simulink model "rfsoc4x2_ospfb_128"  (R2021a)
settings: Solver=VariableStepAuto  StartTime=0.0  StopTime=2048  RelTol=1e-3
undefined symbols (not defined in the file): pfb_coeff_gen_calc
libraries: xbsIndex_r4 x37092, casper_library_delays x737, casper_library_misc x68, xps_library x1
(part 274 of 339)

== system rfsoc4x2_ospfb_128/fft_wideband_real1/fft_biplex_real_4x/biplex_core/fft_stage_3/butterfly_direct/bus_convert ==
  din : Inport
  bussify : Subsystem  AncestorBlock=casper_library_flow_control/bus_create  mask(bus_create){inputNum=16}
      mask prompts: inputNum "Number of inputs:"
      mask init:
      | bus_create_init(gcb,...
      |     'inputNum', inputNum);
  conv1 : Subsystem  AncestorBlock=casper_library_misc/convert_of  mask(convert_of){bit_width_i=21, binary_point_i=18, bit_width_o=18, binary_point_o=17, csp_latency=3, overflow=Wrap, quantization=Round  (unbiased: +/- Inf)}
      mask prompts: bit_width_i "Bit Width In"; binary_point_i "Binary Point In"; bit_width_o "Bit Width Out"; binary_point_o "Binary Point Out"; csp_latency "Latency"; overflow "Overflow Behaviour"; quantization "Quantization Behaviour"
      mask help:
      | Converts from one 2's complement bit-width
      | and/or binary point position to another.
      | Includes underflow/overflow indicator.
      mask init: same as rfsoc4x2_ospfb_128/fft2/fft_direct/butterfly0_0/bus_convert/conv1
      settings: AttributesFormatString=[21,18]->[18,17]
      mask TypeOptions overflow: Wrap | Saturate | Error
      mask TypeOptions quantization: Truncate | Round  (unbiased: +/- Inf) | Round  (unbiased: even values)
  conv10 : Subsystem  AncestorBlock=casper_library_misc/convert_of  mask(convert_of){bit_width_i=21, binary_point_i=18, bit_width_o=18, binary_point_o=17, csp_latency=3, overflow=Wrap, quantization=Round  (unbiased: +/- Inf)}
      mask prompts: bit_width_i "Bit Width In"; binary_point_i "Binary Point In"; bit_width_o "Bit Width Out"; binary_point_o "Binary Point Out"; csp_latency "Latency"; overflow "Overflow Behaviour"; quantization "Quantization Behaviour"
      mask help:
      | Converts from one 2's complement bit-width
      | and/or binary point position to another.
      | Includes underflow/overflow indicator.
      mask init: same as rfsoc4x2_ospfb_128/fft2/fft_direct/butterfly0_0/bus_convert/conv1
      settings: AttributesFormatString=[21,18]->[18,17]
      mask TypeOptions overflow: Wrap | Saturate | Error
      mask TypeOptions quantization: Truncate | Round  (unbiased: +/- Inf) | Round  (unbiased: even values)
  conv11 : Subsystem  AncestorBlock=casper_library_misc/convert_of  mask(convert_of){bit_width_i=21, binary_point_i=18, bit_width_o=18, binary_point_o=17, csp_latency=3, overflow=Wrap, quantization=Round  (unbiased: +/- Inf)}
      mask prompts: bit_width_i "Bit Width In"; binary_point_i "Binary Point In"; bit_width_o "Bit Width Out"; binary_point_o "Binary Point Out"; csp_latency "Latency"; overflow "Overflow Behaviour"; quantization "Quantization Behaviour"
      mask help:
      | Converts from one 2's complement bit-width
      | and/or binary point position to another.
      | Includes underflow/overflow indicator.
      mask init: same as rfsoc4x2_ospfb_128/fft2/fft_direct/butterfly0_0/bus_convert/conv1
      settings: AttributesFormatString=[21,18]->[18,17]
      mask TypeOptions overflow: Wrap | Saturate | Error
      mask TypeOptions quantization: Truncate | Round  (unbiased: +/- Inf) | Round  (unbiased: even values)
  conv12 : Subsystem  AncestorBlock=casper_library_misc/convert_of  mask(convert_of){bit_width_i=21, binary_point_i=18, bit_width_o=18, binary_point_o=17, csp_latency=3, overflow=Wrap, quantization=Round  (unbiased: +/- Inf)}
      mask prompts: bit_width_i "Bit Width In"; binary_point_i "Binary Point In"; bit_width_o "Bit Width Out"; binary_point_o "Binary Point Out"; csp_latency "Latency"; overflow "Overflow Behaviour"; quantization "Quantization Behaviour"
      mask help:
      | Converts from one 2's complement bit-width
      | and/or binary point position to another.
      | Includes underflow/overflow indicator.
      mask init: same as rfsoc4x2_ospfb_128/fft2/fft_direct/butterfly0_0/bus_convert/conv1
      settings: AttributesFormatString=[21,18]->[18,17]
      mask TypeOptions overflow: Wrap | Saturate | Error
      mask TypeOptions quantization: Truncate | Round  (unbiased: +/- Inf) | Round  (unbiased: even values)
  conv13 : Subsystem  AncestorBlock=casper_library_misc/convert_of  mask(convert_of){bit_width_i=21, binary_point_i=18, bit_width_o=18, binary_point_o=17, csp_latency=3, overflow=Wrap, quantization=Round  (unbiased: +/- Inf)}
      mask prompts: bit_width_i "Bit Width In"; binary_point_i "Binary Point In"; bit_width_o "Bit Width Out"; binary_point_o "Binary Point Out"; csp_latency "Latency"; overflow "Overflow Behaviour"; quantization "Quantization Behaviour"
      mask help:
      | Converts from one 2's complement bit-width
      | and/or binary point position to another.
      | Includes underflow/overflow indicator.
      mask init: same as rfsoc4x2_ospfb_128/fft2/fft_direct/butterfly0_0/bus_convert/conv1
      settings: AttributesFormatString=[21,18]->[18,17]
      mask TypeOptions overflow: Wrap | Saturate | Error
      mask TypeOptions quantization: Truncate | Round  (unbiased: +/- Inf) | Round  (unbiased: even values)
  conv14 : Subsystem  AncestorBlock=casper_library_misc/convert_of  mask(convert_of){bit_width_i=21, binary_point_i=18, bit_width_o=18, binary_point_o=17, csp_latency=3, overflow=Wrap, quantization=Round  (unbiased: +/- Inf)}
      mask prompts: bit_width_i "Bit Width In"; binary_point_i "Binary Point In"; bit_width_o "Bit Width Out"; binary_point_o "Binary Point Out"; csp_latency "Latency"; overflow "Overflow Behaviour"; quantization "Quantization Behaviour"
      mask help:
      | Converts from one 2's complement bit-width
      | and/or binary point position to another.
      | Includes underflow/overflow indicator.
      mask init: same as rfsoc4x2_ospfb_128/fft2/fft_direct/butterfly0_0/bus_convert/conv1
      settings: AttributesFormatString=[21,18]->[18,17]
      mask TypeOptions overflow: Wrap | Saturate | Error
      mask TypeOptions quantization: Truncate | Round  (unbiased: +/- Inf) | Round  (unbiased: even values)
  conv15 : Subsystem  AncestorBlock=casper_library_misc/convert_of  mask(convert_of){bit_width_i=21, binary_point_i=18, bit_width_o=18, binary_point_o=17, csp_latency=3, overflow=Wrap, quantization=Round  (unbiased: +/- Inf)}
      mask prompts: bit_width_i "Bit Width In"; binary_point_i "Binary Point In"; bit_width_o "Bit Width Out"; binary_point_o "Binary Point Out"; csp_latency "Latency"; overflow "Overflow Behaviour"; quantization "Quantization Behaviour"
      mask help:
      | Converts from one 2's complement bit-width
      | and/or binary point position to another.
      | Includes underflow/overflow indicator.
      mask init: same as rfsoc4x2_ospfb_128/fft2/fft_direct/butterfly0_0/bus_convert/conv1
      settings: AttributesFormatString=[21,18]->[18,17]
      mask TypeOptions overflow: Wrap | Saturate | Error
      mask TypeOptions quantization: Truncate | Round  (unbiased: +/- Inf) | Round  (unbiased: even values)
  conv16 : Subsystem  AncestorBlock=casper_library_misc/convert_of  mask(convert_of){bit_width_i=21, binary_point_i=18, bit_width_o=18, binary_point_o=17, csp_latency=3, overflow=Wrap, quantization=Round  (unbiased: +/- Inf)}
      mask prompts: bit_width_i "Bit Width In"; binary_point_i "Binary Point In"; bit_width_o "Bit Width Out"; binary_point_o "Binary Point Out"; csp_latency "Latency"; overflow "Overflow Behaviour"; quantization "Quantization Behaviour"
      mask help:
      | Converts from one 2's complement bit-width
      | and/or binary point position to another.
      | Includes underflow/overflow indicator.
      mask init: same as rfsoc4x2_ospfb_128/fft2/fft_direct/butterfly0_0/bus_convert/conv1
      settings: AttributesFormatString=[21,18]->[18,17]
      mask TypeOptions overflow: Wrap | Saturate | Error
      mask TypeOptions quantization: Truncate | Round  (unbiased: +/- Inf) | Round  (unbiased: even values)
  conv2 : Subsystem  AncestorBlock=casper_library_misc/convert_of  mask(convert_of){bit_width_i=21, binary_point_i=18, bit_width_o=18, binary_point_o=17, csp_latency=3, overflow=Wrap, quantization=Round  (unbiased: +/- Inf)}
      mask prompts: bit_width_i "Bit Width In"; binary_point_i "Binary Point In"; bit_width_o "Bit Width Out"; binary_point_o "Binary Point Out"; csp_latency "Latency"; overflow "Overflow Behaviour"; quantization "Quantization Behaviour"
      mask help:
      | Converts from one 2's complement bit-width
      | and/or binary point position to another.
      | Includes underflow/overflow indicator.
      mask init: same as rfsoc4x2_ospfb_128/fft2/fft_direct/butterfly0_0/bus_convert/conv1
      settings: AttributesFormatString=[21,18]->[18,17]
      mask TypeOptions overflow: Wrap | Saturate | Error
      mask TypeOptions quantization: Truncate | Round  (unbiased: +/- Inf) | Round  (unbiased: even values)
  conv3 : Subsystem  AncestorBlock=casper_library_misc/convert_of  mask(convert_of){bit_width_i=21, binary_point_i=18, bit_width_o=18, binary_point_o=17, csp_latency=3, overflow=Wrap, quantization=Round  (unbiased: +/- Inf)}
      mask prompts: bit_width_i "Bit Width In"; binary_point_i "Binary Point In"; bit_width_o "Bit Width Out"; binary_point_o "Binary Point Out"; csp_latency "Latency"; overflow "Overflow Behaviour"; quantization "Quantization Behaviour"
      mask help:
      | Converts from one 2's complement bit-width
      | and/or binary point position to another.
      | Includes underflow/overflow indicator.
      mask init: same as rfsoc4x2_ospfb_128/fft2/fft_direct/butterfly0_0/bus_convert/conv1
      settings: AttributesFormatString=[21,18]->[18,17]
      mask TypeOptions overflow: Wrap | Saturate | Error
      mask TypeOptions quantization: Truncate | Round  (unbiased: +/- Inf) | Round  (unbiased: even values)
  conv4 : Subsystem  AncestorBlock=casper_library_misc/convert_of  mask(convert_of){bit_width_i=21, binary_point_i=18, bit_width_o=18, binary_point_o=17, csp_latency=3, overflow=Wrap, quantization=Round  (unbiased: +/- Inf)}
      mask prompts: bit_width_i "Bit Width In"; binary_point_i "Binary Point In"; bit_width_o "Bit Width Out"; binary_point_o "Binary Point Out"; csp_latency "Latency"; overflow "Overflow Behaviour"; quantization "Quantization Behaviour"
      mask help:
      | Converts from one 2's complement bit-width
      | and/or binary point position to another.
      | Includes underflow/overflow indicator.
      mask init: same as rfsoc4x2_ospfb_128/fft2/fft_direct/butterfly0_0/bus_convert/conv1
      settings: AttributesFormatString=[21,18]->[18,17]
      mask TypeOptions overflow: Wrap | Saturate | Error
      mask TypeOptions quantization: Truncate | Round  (unbiased: +/- Inf) | Round  (unbiased: even values)
  conv5 : Subsystem  AncestorBlock=casper_library_misc/convert_of  mask(convert_of){bit_width_i=21, binary_point_i=18, bit_width_o=18, binary_point_o=17, csp_latency=3, overflow=Wrap, quantization=Round  (unbiased: +/- Inf)}
      mask prompts: bit_width_i "Bit Width In"; binary_point_i "Binary Point In"; bit_width_o "Bit Width Out"; binary_point_o "Binary Point Out"; csp_latency "Latency"; overflow "Overflow Behaviour"; quantization "Quantization Behaviour"
      mask help:
      | Converts from one 2's complement bit-width
      | and/or binary point position to another.
      | Includes underflow/overflow indicator.
      mask init: same as rfsoc4x2_ospfb_128/fft2/fft_direct/butterfly0_0/bus_convert/conv1
      settings: AttributesFormatString=[21,18]->[18,17]
      mask TypeOptions overflow: Wrap | Saturate | Error
      mask TypeOptions quantization: Truncate | Round  (unbiased: +/- Inf) | Round  (unbiased: even values)
  conv6 : Subsystem  AncestorBlock=casper_library_misc/convert_of  mask(convert_of){bit_width_i=21, binary_point_i=18, bit_width_o=18, binary_point_o=17, csp_latency=3, overflow=Wrap, quantization=Round  (unbiased: +/- Inf)}
      mask prompts: bit_width_i "Bit Width In"; binary_point_i "Binary Point In"; bit_width_o "Bit Width Out"; binary_point_o "Binary Point Out"; csp_latency "Latency"; overflow "Overflow Behaviour"; quantization "Quantization Behaviour"
      mask help:
      | Converts from one 2's complement bit-width
      | and/or binary point position to another.
      | Includes underflow/overflow indicator.
      mask init: same as rfsoc4x2_ospfb_128/fft2/fft_direct/butterfly0_0/bus_convert/conv1
      settings: AttributesFormatString=[21,18]->[18,17]
      mask TypeOptions overflow: Wrap | Saturate | Error
      mask TypeOptions quantization: Truncate | Round  (unbiased: +/- Inf) | Round  (unbiased: even values)
  conv7 : Subsystem  AncestorBlock=casper_library_misc/convert_of  mask(convert_of){bit_width_i=21, binary_point_i=18, bit_width_o=18, binary_point_o=17, csp_latency=3, overflow=Wrap, quantization=Round  (unbiased: +/- Inf)}
      mask prompts: bit_width_i "Bit Width In"; binary_point_i "Binary Point In"; bit_width_o "Bit Width Out"; binary_point_o "Binary Point Out"; csp_latency "Latency"; overflow "Overflow Behaviour"; quantization "Quantization Behaviour"
      mask help:
      | Converts from one 2's complement bit-width
      | and/or binary point position to another.
      | Includes underflow/overflow indicator.
      mask init: same as rfsoc4x2_ospfb_128/fft2/fft_direct/butterfly0_0/bus_convert/conv1
      settings: AttributesFormatString=[21,18]->[18,17]
      mask TypeOptions overflow: Wrap | Saturate | Error
      mask TypeOptions quantization: Truncate | Round  (unbiased: +/- Inf) | Round  (unbiased: even values)
  conv8 : Subsystem  AncestorBlock=casper_library_misc/convert_of  mask(convert_of){bit_width_i=21, binary_point_i=18, bit_width_o=18, binary_point_o=17, csp_latency=3, overflow=Wrap, quantization=Round  (unbiased: +/- Inf)}
      mask prompts: bit_width_i "Bit Width In"; binary_point_i "Binary Point In"; bit_width_o "Bit Width Out"; binary_point_o "Binary Point Out"; csp_latency "Latency"; overflow "Overflow Behaviour"; quantization "Quantization Behaviour"
      mask help:
      | Converts from one 2's complement bit-width
      | and/or binary point position to another.
      | Includes underflow/overflow indicator.
      mask init: same as rfsoc4x2_ospfb_128/fft2/fft_direct/butterfly0_0/bus_convert/conv1
      settings: AttributesFormatString=[21,18]->[18,17]
      mask TypeOptions overflow: Wrap | Saturate | Error
      mask TypeOptions quantization: Truncate | Round  (unbiased: +/- Inf) | Round  (unbiased: even values)
  conv9 : Subsystem  AncestorBlock=casper_library_misc/convert_of  mask(convert_of){bit_width_i=21, binary_point_i=18, bit_width_o=18, binary_point_o=17, csp_latency=3, overflow=Wrap, quantization=Round  (unbiased: +/- Inf)}
      mask prompts: bit_width_i "Bit Width In"; binary_point_i "Binary Point In"; bit_width_o "Bit Width Out"; binary_point_o "Binary Point Out"; csp_latency "Latency"; overflow "Overflow Behaviour"; quantization "Quantization Behaviour"
      mask help:
      | Converts from one 2's complement bit-width
      | and/or binary point position to another.
      | Includes underflow/overflow indicator.
      mask init: same as rfsoc4x2_ospfb_128/fft2/fft_direct/butterfly0_0/bus_convert/conv1
      settings: AttributesFormatString=[21,18]->[18,17]
      mask TypeOptions overflow: Wrap | Saturate | Error
      mask TypeOptions quantization: Truncate | Round  (unbiased: +/- Inf) | Round  (unbiased: even values)
  debus : Subsystem  AncestorBlock=casper_library_flow_control/bus_expand  mask(bus_expand){mode=divisions of arbitrary size, outputNum=2, outputWidth=[21 21 21 21 21 21 21 21 21 21 21 21 21 21 21 21], outputBinaryPt=[18 18 18 18 18 18 18 18 18 18 18 18 18 18 18 18], outputArithmeticType=[1 1 1 1 1 1 1 1 1 1 1 1 1 1 1 1], show_format=on, outputToWorkspace=off, variablePrefix=, outputToModelAsWell=on}
      mask prompts: outputNum "Number of outputs:"; outputWidth "Output width:"; outputBinaryPt "Output binary point position:"; outputArithmeticType "Output arithmetic type (ufix=0, fix=1, bool=2):"; show_format "Print format string?"; outputToWorkspace "Output to workspace?"; variablePrefix "Variable name prefix:"; outputToModelAsWell "Output to model as well?"
      mask help:
      | Expands a 'bus' made using a bus_create or Xilinx
      | concat block.
      | The input will be divided into the specified number
      | of outputs with the specified arithmetic types.
      | Divisions are made from most significant bit.
      mask init: same as rfsoc4x2_ospfb_128/bus_expand1
      settings: AttributesFormatString=16 outputs: f21.18,f21.18,f21.18,f21.18,f21.18,f21.18,f21.18,f21.18,f21.18,f21.18,f21.18,f21.18,f21.18,f21.18,f21.18,f21.18,
      mask TypeOptions mode: divisions of equal size | divisions of arbitrary size
      mask Callback mode: %bus_expand_callback();
      mask Callback outputWidth: %bus_expand_callback();
      mask Callback outputToWorkspace: %bus_expand_callback();
  of_bussify : Subsystem  AncestorBlock=casper_library_flow_control/bus_create  mask(bus_create){inputNum=16}
      mask prompts: inputNum "Number of inputs:"
      mask init:
      | bus_create_init(gcb,...
      |     'inputNum', inputNum);
  dout : Outport
  overflow : Outport  Port=2
  wires:
  of_bussify/1(bus_out) -> overflow/1
  bussify/1(bus_out) -> dout/1
  conv16/2(of) -> of_bussify/16(in16)
  conv15/2(of) -> of_bussify/15(in15)
  conv14/2(of) -> of_bussify/14(in14)
  conv13/2(of) -> of_bussify/13(in13)
  conv12/2(of) -> of_bussify/12(in12)
  conv11/2(of) -> of_bussify/11(in11)
  conv10/2(of) -> of_bussify/10(in10)
  conv9/2(of) -> of_bussify/9(in9)
  conv8/2(of) -> of_bussify/8(in8)
  conv7/2(of) -> of_bussify/7(in7)
  conv6/2(of) -> of_bussify/6(in6)
  conv5/2(of) -> of_bussify/5(in5)
  conv4/2(of) -> of_bussify/4(in4)
  conv3/2(of) -> of_bussify/3(in3)
  conv2/2(of) -> of_bussify/2(in2)
  conv1/2(of) -> of_bussify/1(in1)
  conv16/1(dout) -> bussify/16(in16)
  conv15/1(dout) -> bussify/15(in15)
  conv14/1(dout) -> bussify/14(in14)
  conv13/1(dout) -> bussify/13(in13)
  conv12/1(dout) -> bussify/12(in12)
  conv11/1(dout) -> bussify/11(in11)
  conv10/1(dout) -> bussify/10(in10)
  conv9/1(dout) -> bussify/9(in9)
  conv8/1(dout) -> bussify/8(in8)
  conv7/1(dout) -> bussify/7(in7)
  conv6/1(dout) -> bussify/6(in6)
  conv5/1(dout) -> bussify/5(in5)
  conv4/1(dout) -> bussify/4(in4)
  conv3/1(dout) -> bussify/3(in3)
  conv2/1(dout) -> bussify/2(in2)
  conv1/1(dout) -> bussify/1(in1)
  debus/16(lsb_out1) -> conv16/1(din)
  debus/15(out2) -> conv15/1(din)
  debus/14(out3) -> conv14/1(din)
  debus/13(out4) -> conv13/1(din)
  debus/12(out5) -> conv12/1(din)
  debus/11(out6) -> conv11/1(din)
  debus/10(out7) -> conv10/1(din)
  debus/9(out8) -> conv9/1(din)
  debus/8(out9) -> conv8/1(din)
  debus/7(out10) -> conv7/1(din)
  debus/6(out11) -> conv6/1(din)
  debus/5(out12) -> conv5/1(din)
  debus/4(out13) -> conv4/1(din)
  debus/3(out14) -> conv3/1(din)
  debus/2(out15) -> conv2/1(din)
  debus/1(msb_out16) -> conv1/1(din)
  din/1 -> debus/1(bus_in)

== system rfsoc4x2_ospfb_128/fft_wideband_real1/fft_biplex_real_4x/biplex_core/fft_stage_3/butterfly_direct/bus_expand ==
  bus_in : Inport
  reinterpret1 : xbsIndex_r4/Reinterpret  force_arith_type=on  arith_type=Unsigned  force_bin_pt=on  bin_pt=0  block_type=reinterpret
  reinterpret2 : xbsIndex_r4/Reinterpret  force_arith_type=on  arith_type=Unsigned  force_bin_pt=on  bin_pt=0  block_type=reinterpret
  slice1 : xbsIndex_r4/Slice  nbits=144  boolean_output=off  mode=Upper Bit Location + Width  bit1=-144  base1=MSB of Input  bit0=0  base0=LSB of Input  dbl_ovrd=off  block_type=slice
  slice2 : xbsIndex_r4/Slice  nbits=144  boolean_output=off  mode=Upper Bit Location + Width  bit1=0  base1=MSB of Input  bit0=0  base0=LSB of Input  dbl_ovrd=off  block_type=slice
  msb_out2 : Outport  VectorParamsAs1DForOutWhenUnconnected=off
  lsb_out1 : Outport  Port=2  VectorParamsAs1DForOutWhenUnconnected=off
  wires:
  reinterpret1/1 -> lsb_out1/1
  slice1/1 -> reinterpret1/1
  reinterpret2/1 -> msb_out2/1
  slice2/1 -> reinterpret2/1
  bus_in/1 -> slice1/1, slice2/1

== system rfsoc4x2_ospfb_128/fft_wideband_real1/fft_biplex_real_4x/biplex_core/fft_stage_3/butterfly_direct/bus_norm0 ==
  din : Inport
  bussify : Subsystem  AncestorBlock=casper_library_flow_control/bus_create  mask(bus_create){inputNum=16}
      mask prompts: inputNum "Number of inputs:"
      mask init:
      | bus_create_init(gcb,...
      |     'inputNum', inputNum);
  conv{1..16} (16 alike) : xbsIndex_r4/Convert  gui_display_data_type=Fixed-point  arith_type="Signed  (2's comp)"  n_bits=21  bin_pt=18  float_type=Single  exp_bits=8  fraction_bits=24  quantization=Truncate  overflow=Wrap  en=off  latency=0  pipeline=on  dbl_ovrd=off  block_type=convert
  debus : Subsystem  AncestorBlock=casper_library_flow_control/bus_expand  mask(bus_expand){mode=divisions of arbitrary size, outputNum=2, outputWidth=[20 20 20 20 20 20 20 20 20 20 20 20 20 20 20 20], outputBinaryPt=[17 17 17 17 17 17 17 17 17 17 17 17 17 17 17 17], outputArithmeticType=[1 1 1 1 1 1 1 1 1 1 1 1 1 1 1 1], show_format=on, outputToWorkspace=off, variablePrefix=, outputToModelAsWell=on}
      mask prompts: outputNum "Number of outputs:"; outputWidth "Output width:"; outputBinaryPt "Output binary point position:"; outputArithmeticType "Output arithmetic type (ufix=0, fix=1, bool=2):"; show_format "Print format string?"; outputToWorkspace "Output to workspace?"; variablePrefix "Variable name prefix:"; outputToModelAsWell "Output to model as well?"
      mask help:
      | Expands a 'bus' made using a bus_create or Xilinx
      | concat block.
      | The input will be divided into the specified number
      | of outputs with the specified arithmetic types.
      | Divisions are made from most significant bit.
      mask init: same as rfsoc4x2_ospfb_128/bus_expand1
      settings: AttributesFormatString=16 outputs: f20.17,f20.17,f20.17,f20.17,f20.17,f20.17,f20.17,f20.17,f20.17,f20.17,f20.17,f20.17,f20.17,f20.17,f20.17,f20.17,
      mask TypeOptions mode: divisions of equal size | divisions of arbitrary size
      mask Callback mode: %bus_expand_callback();
      mask Callback outputWidth: %bus_expand_callback();
      mask Callback outputToWorkspace: %bus_expand_callback();
  dout : Outport
  wires:
  bussify/1(bus_out) -> dout/1
  conv16/1 -> bussify/16(in16)
  conv15/1 -> bussify/15(in15)
  conv14/1 -> bussify/14(in14)
  conv13/1 -> bussify/13(in13)
  conv12/1 -> bussify/12(in12)
  conv11/1 -> bussify/11(in11)
  conv10/1 -> bussify/10(in10)
  conv9/1 -> bussify/9(in9)
  conv8/1 -> bussify/8(in8)
  conv7/1 -> bussify/7(in7)
  conv6/1 -> bussify/6(in6)
  conv5/1 -> bussify/5(in5)
  conv4/1 -> bussify/4(in4)
  conv3/1 -> bussify/3(in3)
  conv2/1 -> bussify/2(in2)
  conv1/1 -> bussify/1(in1)
  debus/16(lsb_out1) -> conv16/1
  debus/15(out2) -> conv15/1
  debus/14(out3) -> conv14/1
  debus/13(out4) -> conv13/1
  debus/12(out5) -> conv12/1
  debus/11(out6) -> conv11/1
  debus/10(out7) -> conv10/1
  debus/9(out8) -> conv9/1
  debus/8(out9) -> conv8/1
  debus/7(out10) -> conv7/1
  debus/6(out11) -> conv6/1
  debus/5(out12) -> conv5/1
  debus/4(out13) -> conv4/1
  debus/3(out14) -> conv3/1
  debus/2(out15) -> conv2/1
  debus/1(msb_out16) -> conv1/1
  din/1 -> debus/1(bus_in)

== system rfsoc4x2_ospfb_128/fft_wideband_real1/fft_biplex_real_4x/biplex_core/fft_stage_3/butterfly_direct/bus_norm1 ==
  din : Inport
  bussify : Subsystem  AncestorBlock=casper_library_flow_control/bus_create  mask(bus_create){inputNum=16}
      mask prompts: inputNum "Number of inputs:"
      mask init:
      | bus_create_init(gcb,...
      |     'inputNum', inputNum);
  conv{1..16} (16 alike) : xbsIndex_r4/Convert  gui_display_data_type=Fixed-point  arith_type="Signed  (2's comp)"  n_bits=21  bin_pt=18  float_type=Single  exp_bits=8  fraction_bits=24  quantization=Truncate  overflow=Wrap  en=off  latency=0  pipeline=on  dbl_ovrd=off  block_type=convert
  debus : Subsystem  AncestorBlock=casper_library_flow_control/bus_expand  mask(bus_expand){mode=divisions of arbitrary size, outputNum=2, outputWidth=[20 20 20 20 20 20 20 20 20 20 20 20 20 20 20 20], outputBinaryPt=[18 18 18 18 18 18 18 18 18 18 18 18 18 18 18 18], outputArithmeticType=[1 1 1 1 1 1 1 1 1 1 1 1 1 1 1 1], show_format=on, outputToWorkspace=off, variablePrefix=, outputToModelAsWell=on}
      mask prompts: outputNum "Number of outputs:"; outputWidth "Output width:"; outputBinaryPt "Output binary point position:"; outputArithmeticType "Output arithmetic type (ufix=0, fix=1, bool=2):"; show_format "Print format string?"; outputToWorkspace "Output to workspace?"; variablePrefix "Variable name prefix:"; outputToModelAsWell "Output to model as well?"
      mask help:
      | Expands a 'bus' made using a bus_create or Xilinx
      | concat block.
      | The input will be divided into the specified number
      | of outputs with the specified arithmetic types.
      | Divisions are made from most significant bit.
      mask init: same as rfsoc4x2_ospfb_128/bus_expand1
      settings: AttributesFormatString=16 outputs: f20.18,f20.18,f20.18,f20.18,f20.18,f20.18,f20.18,f20.18,f20.18,f20.18,f20.18,f20.18,f20.18,f20.18,f20.18,f20.18,
      mask TypeOptions mode: divisions of equal size | divisions of arbitrary size
      mask Callback mode: %bus_expand_callback();
      mask Callback outputWidth: %bus_expand_callback();
      mask Callback outputToWorkspace: %bus_expand_callback();
  dout : Outport
  wires:
  bussify/1(bus_out) -> dout/1
  conv16/1 -> bussify/16(in16)
  conv15/1 -> bussify/15(in15)
  conv14/1 -> bussify/14(in14)
  conv13/1 -> bussify/13(in13)
  conv12/1 -> bussify/12(in12)
  conv11/1 -> bussify/11(in11)
  conv10/1 -> bussify/10(in10)
  conv9/1 -> bussify/9(in9)
  conv8/1 -> bussify/8(in8)
  conv7/1 -> bussify/7(in7)
  conv6/1 -> bussify/6(in6)
  conv5/1 -> bussify/5(in5)
  conv4/1 -> bussify/4(in4)
  conv3/1 -> bussify/3(in3)
  conv2/1 -> bussify/2(in2)
  conv1/1 -> bussify/1(in1)
  debus/16(lsb_out1) -> conv16/1
  debus/15(out2) -> conv15/1
  debus/14(out3) -> conv14/1
  debus/13(out4) -> conv13/1
  debus/12(out5) -> conv12/1
  debus/11(out6) -> conv11/1
  debus/10(out7) -> conv10/1
  debus/9(out8) -> conv9/1
  debus/8(out9) -> conv8/1
  debus/7(out10) -> conv7/1
  debus/6(out11) -> conv6/1
  debus/5(out12) -> conv5/1
  debus/4(out13) -> conv4/1
  debus/3(out14) -> conv3/1
  debus/2(out15) -> conv2/1
  debus/1(msb_out16) -> conv1/1
  din/1 -> debus/1(bus_in)

== system rfsoc4x2_ospfb_128/fft_wideband_real1/fft_biplex_real_4x/biplex_core/fft_stage_3/butterfly_direct/bus_relational ==
  a : Inport
  b : Inport  Port=2
  a_debus : Subsystem  AncestorBlock=casper_library_flow_control/bus_expand  mask(bus_expand){mode=divisions of arbitrary size, outputNum=2, outputWidth=[4], outputBinaryPt=[0], outputArithmeticType=[0], show_format=on, outputToWorkspace=off, variablePrefix=, outputToModelAsWell=on}
      mask prompts: outputNum "Number of outputs:"; outputWidth "Output width:"; outputBinaryPt "Output binary point position:"; outputArithmeticType "Output arithmetic type (ufix=0, fix=1, bool=2):"; show_format "Print format string?"; outputToWorkspace "Output to workspace?"; variablePrefix "Variable name prefix:"; outputToModelAsWell "Output to model as well?"
      mask help:
      | Expands a 'bus' made using a bus_create or Xilinx
      | concat block.
      | The input will be divided into the specified number
      | of outputs with the specified arithmetic types.
      | Divisions are made from most significant bit.
      mask init: same as rfsoc4x2_ospfb_128/bus_expand1
      settings: AttributesFormatString=1 outputs: uf4.0,
      mask TypeOptions mode: divisions of equal size | divisions of arbitrary size
      mask Callback mode: %bus_expand_callback();
      mask Callback outputWidth: %bus_expand_callback();
      mask Callback outputToWorkspace: %bus_expand_callback();
  b_debus : Subsystem  AncestorBlock=casper_library_flow_control/bus_expand  mask(bus_expand){mode=divisions of arbitrary size, outputNum=2, outputWidth=[4  4  4  4], outputBinaryPt=[0  0  0  0], outputArithmeticType=[0  0  0  0], show_format=on, outputToWorkspace=off, variablePrefix=, outputToModelAsWell=on}
      mask prompts: outputNum "Number of outputs:"; outputWidth "Output width:"; outputBinaryPt "Output binary point position:"; outputArithmeticType "Output arithmetic type (ufix=0, fix=1, bool=2):"; show_format "Print format string?"; outputToWorkspace "Output to workspace?"; variablePrefix "Variable name prefix:"; outputToModelAsWell "Output to model as well?"
      mask help:
      | Expands a 'bus' made using a bus_create or Xilinx
      | concat block.
      | The input will be divided into the specified number
      | of outputs with the specified arithmetic types.
      | Divisions are made from most significant bit.
      mask init: same as rfsoc4x2_ospfb_128/bus_expand1
      settings: AttributesFormatString=4 outputs: uf4.0,uf4.0,uf4.0,uf4.0,
      mask TypeOptions mode: divisions of equal size | divisions of arbitrary size
      mask Callback mode: %bus_expand_callback();
      mask Callback outputWidth: %bus_expand_callback();
      mask Callback outputToWorkspace: %bus_expand_callback();
  bussify : Subsystem  AncestorBlock=casper_library_flow_control/bus_create  mask(bus_create){inputNum=4}
      mask prompts: inputNum "Number of inputs:"
      mask init:
      | bus_create_init(gcb,...
      |     'inputNum', inputNum);
  relational{1..4} (4 alike) : xbsIndex_r4/Relational  mode=a!=b  op_type=Bool  en=off  latency=1  dbl_ovrd=off  block_type=relational
  a!=b : Outport
  wires:
  bussify/1(bus_out) -> a!=b/1
  relational4/1 -> bussify/4(in4)
  relational3/1 -> bussify/3(in3)
  relational2/1 -> bussify/2(in2)
  relational1/1 -> bussify/1(in1)
  b_debus/4(lsb_out1) -> relational4/2
  b_debus/3(out2) -> relational3/2
  b_debus/2(out3) -> relational2/2
  b_debus/1(msb_out4) -> relational1/2
  a_debus/1(msb_lsb_out1) -> relational4/1, relational3/1, relational2/1, relational1/1
  b/1 -> b_debus/1(bus_in)
  a/1 -> a_debus/1(bus_in)

== system rfsoc4x2_ospfb_128/fft_wideband_real1/fft_biplex_real_4x/biplex_core/fft_stage_3/butterfly_direct/bus_scale ==
  din : Inport
  bussify : Subsystem  AncestorBlock=casper_library_flow_control/bus_create  mask(bus_create){inputNum=16}
      mask prompts: inputNum "Number of inputs:"
      mask init:
      | bus_create_init(gcb,...
      |     'inputNum', inputNum);
  debus : Subsystem  AncestorBlock=casper_library_flow_control/bus_expand  mask(bus_expand){mode=divisions of arbitrary size, outputNum=2, outputWidth=[20 20 20 20 20 20 20 20 20 20 20 20 20 20 20 20], outputBinaryPt=[17 17 17 17 17 17 17 17 17 17 17 17 17 17 17 17], outputArithmeticType=[1 1 1 1 1 1 1 1 1 1 1 1 1 1 1 1], show_format=on, outputToWorkspace=off, variablePrefix=, outputToModelAsWell=on}
      mask prompts: outputNum "Number of outputs:"; outputWidth "Output width:"; outputBinaryPt "Output binary point position:"; outputArithmeticType "Output arithmetic type (ufix=0, fix=1, bool=2):"; show_format "Print format string?"; outputToWorkspace "Output to workspace?"; variablePrefix "Variable name prefix:"; outputToModelAsWell "Output to model as well?"
      mask help:
      | Expands a 'bus' made using a bus_create or Xilinx
      | concat block.
      | The input will be divided into the specified number
      | of outputs with the specified arithmetic types.
      | Divisions are made from most significant bit.
      mask init: same as rfsoc4x2_ospfb_128/bus_expand1
      settings: AttributesFormatString=16 outputs: f20.17,f20.17,f20.17,f20.17,f20.17,f20.17,f20.17,f20.17,f20.17,f20.17,f20.17,f20.17,f20.17,f20.17,f20.17,f20.17,
      mask TypeOptions mode: divisions of equal size | divisions of arbitrary size
      mask Callback mode: %bus_expand_callback();
      mask Callback outputWidth: %bus_expand_callback();
      mask Callback outputToWorkspace: %bus_expand_callback();
  scale{1..16} (16 alike) : xbsIndex_r4/Scale  scale_factor=-1  dbl_ovrd=off  block_type=scale
  dout : Outport
  wires:
  bussify/1(bus_out) -> dout/1
  scale16/1 -> bussify/16(in16)
  scale15/1 -> bussify/15(in15)
  scale14/1 -> bussify/14(in14)
  scale13/1 -> bussify/13(in13)
  scale12/1 -> bussify/12(in12)
  scale11/1 -> bussify/11(in11)
  scale10/1 -> bussify/10(in10)
  scale9/1 -> bussify/9(in9)
  scale8/1 -> bussify/8(in8)
  scale7/1 -> bussify/7(in7)
  scale6/1 -> bussify/6(in6)
  scale5/1 -> bussify/5(in5)
  scale4/1 -> bussify/4(in4)
  scale3/1 -> bussify/3(in3)
  scale2/1 -> bussify/2(in2)
  scale1/1 -> bussify/1(in1)
  debus/16(lsb_out1) -> scale16/1
  debus/15(out2) -> scale15/1
  debus/14(out3) -> scale14/1
  debus/13(out4) -> scale13/1
  debus/12(out5) -> scale12/1
  debus/11(out6) -> scale11/1
  debus/10(out7) -> scale10/1
  debus/9(out8) -> scale9/1
  debus/8(out9) -> scale8/1
  debus/7(out10) -> scale7/1
  debus/6(out11) -> scale6/1
  debus/5(out12) -> scale5/1
  debus/4(out13) -> scale4/1
  debus/3(out14) -> scale3/1
  debus/2(out15) -> scale2/1
  debus/1(msb_out16) -> scale1/1
  din/1 -> debus/1(bus_in)

== system rfsoc4x2_ospfb_128/fft_wideband_real1/fft_biplex_real_4x/biplex_core/fft_stage_3/butterfly_direct/bus_sub ==
  a : Inport
  b : Inport  Port=2
  a_debus : Subsystem  AncestorBlock=casper_library_flow_control/bus_expand  mask(bus_expand){mode=divisions of arbitrary size, outputNum=2, outputWidth=[18  18  18  18  18  18  18  18], outputBinaryPt=[17  17  17  17  17  17  17  17], outputArithmeticType=[1  1  1  1  1  1  1  1], show_format=on, outputToWorkspace=off, variablePrefix=, outputToModelAsWell=on}
      mask prompts: outputNum "Number of outputs:"; outputWidth "Output width:"; outputBinaryPt "Output binary point position:"; outputArithmeticType "Output arithmetic type (ufix=0, fix=1, bool=2):"; show_format "Print format string?"; outputToWorkspace "Output to workspace?"; variablePrefix "Variable name prefix:"; outputToModelAsWell "Output to model as well?"
      mask help:
      | Expands a 'bus' made using a bus_create or Xilinx
      | concat block.
      | The input will be divided into the specified number
      | of outputs with the specified arithmetic types.
      | Divisions are made from most significant bit.
      mask init: same as rfsoc4x2_ospfb_128/bus_expand1
      settings: AttributesFormatString=8 outputs: f18.17,f18.17,f18.17,f18.17,f18.17,f18.17,f18.17,f18.17,
      mask TypeOptions mode: divisions of equal size | divisions of arbitrary size
      mask Callback mode: %bus_expand_callback();
      mask Callback outputWidth: %bus_expand_callback();
      mask Callback outputToWorkspace: %bus_expand_callback();
  addsub{1..8} (8 alike) : xbsIndex_r4/AddSub  mode=Subtraction  use_carryin=off  use_carryout=off  en=off  latency=1  precision=User Defined  arith_type="Signed  (2's comp)"  n_bits=20  bin_pt=17  quantization=Truncate  overflow=Wrap  use_behavioral_HDL=on  hw_selection=Fabric  pipelined=on  dbl_ovrd=off  block_type=addsub
  b_debus : Subsystem  AncestorBlock=casper_library_flow_control/bus_expand  mask(bus_expand){mode=divisions of arbitrary size, outputNum=2, outputWidth=[19  19  19  19  19  19  19  19], outputBinaryPt=[17  17  17  17  17  17  17  17], outputArithmeticType=[1  1  1  1  1  1  1  1], show_format=on, outputToWorkspace=off, variablePrefix=, outputToModelAsWell=on}
      mask prompts: outputNum "Number of outputs:"; outputWidth "Output width:"; outputBinaryPt "Output binary point position:"; outputArithmeticType "Output arithmetic type (ufix=0, fix=1, bool=2):"; show_format "Print format string?"; outputToWorkspace "Output to workspace?"; variablePrefix "Variable name prefix:"; outputToModelAsWell "Output to model as well?"
      mask help:
      | Expands a 'bus' made using a bus_create or Xilinx
      | concat block.
      | The input will be divided into the specified number
      | of outputs with the specified arithmetic types.
      | Divisions are made from most significant bit.
      mask init: same as rfsoc4x2_ospfb_128/bus_expand1
      settings: AttributesFormatString=8 outputs: f19.17,f19.17,f19.17,f19.17,f19.17,f19.17,f19.17,f19.17,
      mask TypeOptions mode: divisions of equal size | divisions of arbitrary size
      mask Callback mode: %bus_expand_callback();
      mask Callback outputWidth: %bus_expand_callback();
      mask Callback outputToWorkspace: %bus_expand_callback();
  op_bussify : Subsystem  AncestorBlock=casper_library_flow_control/bus_create  mask(bus_create){inputNum=8}
      mask prompts: inputNum "Number of inputs:"
      mask init:
      | bus_create_init(gcb,...
      |     'inputNum', inputNum);
  dout : Outport
  wires:
  op_bussify/1(bus_out) -> dout/1
  addsub8/1 -> op_bussify/8(in8)
  addsub7/1 -> op_bussify/7(in7)
  addsub6/1 -> op_bussify/6(in6)
  addsub5/1 -> op_bussify/5(in5)
  addsub4/1 -> op_bussify/4(in4)
  addsub3/1 -> op_bussify/3(in3)
  addsub2/1 -> op_bussify/2(in2)
  addsub1/1 -> op_bussify/1(in1)
  b_debus/8(lsb_out1) -> addsub8/2
  a_debus/8(lsb_out1) -> addsub8/1
  b_debus/7(out2) -> addsub7/2
  a_debus/7(out2) -> addsub7/1
  b_debus/6(out3) -> addsub6/2
  a_debus/6(out3) -> addsub6/1
  b_debus/5(out4) -> addsub5/2
  a_debus/5(out4) -> addsub5/1
  b_debus/4(out5) -> addsub4/2
  a_debus/4(out5) -> addsub4/1
  b_debus/3(out6) -> addsub3/2
  a_debus/3(out6) -> addsub3/1
  b_debus/2(out7) -> addsub2/2
  a_debus/2(out7) -> addsub2/1
  b_debus/1(msb_out8) -> addsub1/2
  a_debus/1(msb_out8) -> addsub1/1
  b/1 -> b_debus/1(bus_in)
  a/1 -> a_debus/1(bus_in)

== system rfsoc4x2_ospfb_128/fft_wideband_real1/fft_biplex_real_4x/biplex_core/fft_stage_3/butterfly_direct/munge ==
  din : Inport
  join : Subsystem  AncestorBlock=casper_library_flow_control/bus_create  mask(bus_create){inputNum=8}
      mask prompts: inputNum "Number of inputs:"
      mask init:
      | bus_create_init(gcb,...
      |     'inputNum', inputNum);
  reinterpret : xbsIndex_r4/Reinterpret  force_arith_type=on  arith_type=Unsigned  force_bin_pt=on  bin_pt=0  block_type=reinterpret
  reinterpret_out : xbsIndex_r4/Reinterpret  force_arith_type=on  arith_type=Unsigned  force_bin_pt=on  bin_pt=0  block_type=reinterpret
  split : Subsystem  AncestorBlock=casper_library_flow_control/bus_expand  mask(bus_expand){mode=divisions of arbitrary size, outputNum=8, outputWidth=[2 2 2 2 2 2 2 2], outputBinaryPt=[0 0 0 0 0 0 0 0], outputArithmeticType=[0 0 0 0 0 0 0 0], show_format=off, outputToWorkspace=off, variablePrefix=out, outputToModelAsWell=on}
      mask prompts: outputNum "Number of outputs:"; outputWidth "Output width:"; outputBinaryPt "Output binary point position:"; outputArithmeticType "Output arithmetic type (ufix=0, fix=1, bool=2):"; show_format "Print format string?"; outputToWorkspace "Output to workspace?"; variablePrefix "Variable name prefix:"; outputToModelAsWell "Output to model as well?"
      mask help:
      | Expands a 'bus' made using a bus_create or Xilinx
      | concat block.
      | The input will be divided into the specified number
      | of outputs with the specified arithmetic types.
      | Divisions are made from most significant bit.
      mask init: same as rfsoc4x2_ospfb_128/bus_expand1
      settings: AttributesFormatString=8 outputs
      mask TypeOptions mode: divisions of equal size | divisions of arbitrary size
      mask Callback mode: %bus_expand_callback();
      mask Callback outputWidth: %bus_expand_callback();
      mask Callback outputToWorkspace: %bus_expand_callback();
  dout : Outport
  wires:
  split/8(lsb_out1) -> join/8(in8)
  split/4(out5) -> join/7(in7)
  split/7(out2) -> join/6(in6)
  split/3(out6) -> join/5(in5)
  split/6(out3) -> join/4(in4)
  split/2(out7) -> join/3(in3)
  split/5(out4) -> join/2(in2)
  split/1(msb_out8) -> join/1(in1)
  join/1(bus_out) -> reinterpret_out/1
  reinterpret/1 -> split/1(bus_in)
  din/1 -> reinterpret/1
  reinterpret_out/1 -> dout/1

== system rfsoc4x2_ospfb_128/fft_wideband_real1/fft_biplex_real_4x/biplex_core/fft_stage_3/butterfly_direct/mux ==
  sel : Inport
  d0 : Inport  Port=2
  d1 : Inport  Port=3
  d_bussify : Subsystem  AncestorBlock=casper_library_flow_control/bus_create  mask(bus_create){inputNum=16}
      mask prompts: inputNum "Number of inputs:"
      mask init:
      | bus_create_init(gcb,...
      |     'inputNum', inputNum);
  expand0 : Subsystem  AncestorBlock=casper_library_flow_control/bus_expand  mask(bus_expand){mode=divisions of arbitrary size, outputNum=2, outputWidth=[21 21 21 21 21 21 21 21 21 21 21 21 21 21 21 21], outputBinaryPt=[0  0  0  0  0  0  0  0  0  0  0  0  0  0  0  0], outputArithmeticType=[0  0  0  0  0  0  0  0  0  0  0  0  0  0  0  0], show_format=on, outputToWorkspace=off, variablePrefix=, outputToModelAsWell=on}
      mask prompts: outputNum "Number of outputs:"; outputWidth "Output width:"; outputBinaryPt "Output binary point position:"; outputArithmeticType "Output arithmetic type (ufix=0, fix=1, bool=2):"; show_format "Print format string?"; outputToWorkspace "Output to workspace?"; variablePrefix "Variable name prefix:"; outputToModelAsWell "Output to model as well?"
      mask help:
      | Expands a 'bus' made using a bus_create or Xilinx
      | concat block.
      | The input will be divided into the specified number
      | of outputs with the specified arithmetic types.
      | Divisions are made from most significant bit.
      mask init: same as rfsoc4x2_ospfb_128/bus_expand1
      settings: AttributesFormatString=16 outputs: uf21.0,uf21.0,uf21.0,uf21.0,uf21.0,uf21.0,uf21.0,uf21.0,uf21.0,uf21.0,uf21.0,uf21.0,uf21.0,uf21.0,uf21.0,uf21.0,
      mask TypeOptions mode: divisions of equal size | divisions of arbitrary size
      mask Callback mode: %bus_expand_callback();
      mask Callback outputWidth: %bus_expand_callback();
      mask Callback outputToWorkspace: %bus_expand_callback();
  expand1 : Subsystem  AncestorBlock=casper_library_flow_control/bus_expand  mask(bus_expand){mode=divisions of arbitrary size, outputNum=2, outputWidth=[21 21 21 21 21 21 21 21 21 21 21 21 21 21 21 21], outputBinaryPt=[0  0  0  0  0  0  0  0  0  0  0  0  0  0  0  0], outputArithmeticType=[0  0  0  0  0  0  0  0  0  0  0  0  0  0  0  0], show_format=on, outputToWorkspace=off, variablePrefix=, outputToModelAsWell=on}
      mask prompts: outputNum "Number of outputs:"; outputWidth "Output width:"; outputBinaryPt "Output binary point position:"; outputArithmeticType "Output arithmetic type (ufix=0, fix=1, bool=2):"; show_format "Print format string?"; outputToWorkspace "Output to workspace?"; variablePrefix "Variable name prefix:"; outputToModelAsWell "Output to model as well?"
      mask help:
      | Expands a 'bus' made using a bus_create or Xilinx
      | concat block.
      | The input will be divided into the specified number
      | of outputs with the specified arithmetic types.
      | Divisions are made from most significant bit.
      mask init: same as rfsoc4x2_ospfb_128/bus_expand1
      settings: AttributesFormatString=16 outputs: uf21.0,uf21.0,uf21.0,uf21.0,uf21.0,uf21.0,uf21.0,uf21.0,uf21.0,uf21.0,uf21.0,uf21.0,uf21.0,uf21.0,uf21.0,uf21.0,
      mask TypeOptions mode: divisions of equal size | divisions of arbitrary size
      mask Callback mode: %bus_expand_callback();
      mask Callback outputWidth: %bus_expand_callback();
      mask Callback outputToWorkspace: %bus_expand_callback();
  mux{0..15} (16 alike) : xbsIndex_r4/Mux  inputs=2  en=off  latency=1  precision=Full  arith_type=Unsigned  n_bits=16  bin_pt=14  quantization=Truncate  overflow=Wrap  dbl_ovrd=off  block_type=mux
  sel_expand : Subsystem  AncestorBlock=casper_library_flow_control/bus_expand  mask(bus_expand){mode=divisions of equal size, outputNum=16, outputWidth=1, outputBinaryPt=0, outputArithmeticType=0, show_format=on, outputToWorkspace=off, variablePrefix=, outputToModelAsWell=on}
      mask prompts: outputNum "Number of outputs:"; outputWidth "Output width:"; outputBinaryPt "Output binary point position:"; outputArithmeticType "Output arithmetic type (ufix=0, fix=1, bool=2):"; show_format "Print format string?"; outputToWorkspace "Output to workspace?"; variablePrefix "Variable name prefix:"; outputToModelAsWell "Output to model as well?"
      mask help:
      | Expands a 'bus' made using a bus_create or Xilinx
      | concat block.
      | The input will be divided into the specified number
      | of outputs with the specified arithmetic types.
      | Divisions are made from most significant bit.
      mask init: same as rfsoc4x2_ospfb_128/bus_expand1
      settings: AttributesFormatString=16 outputs: uf1.0,uf1.0,uf1.0,uf1.0,uf1.0,uf1.0,uf1.0,uf1.0,uf1.0,uf1.0,uf1.0,uf1.0,uf1.0,uf1.0,uf1.0,uf1.0,
      mask TypeOptions mode: divisions of equal size | divisions of arbitrary size
      mask Callback mode: %bus_expand_callback();
      mask Callback outputWidth: %bus_expand_callback();
      mask Callback outputToWorkspace: %bus_expand_callback();
  out : Outport
  wires:
  d_bussify/1(bus_out) -> out/1
  mux15/1 -> d_bussify/16(in16)
  mux14/1 -> d_bussify/15(in15)
  mux13/1 -> d_bussify/14(in14)
  mux12/1 -> d_bussify/13(in13)
  mux11/1 -> d_bussify/12(in12)
  mux10/1 -> d_bussify/11(in11)
  mux9/1 -> d_bussify/10(in10)
  mux8/1 -> d_bussify/9(in9)
  mux7/1 -> d_bussify/8(in8)
  mux6/1 -> d_bussify/7(in7)
  mux5/1 -> d_bussify/6(in6)
  mux4/1 -> d_bussify/5(in5)
  mux3/1 -> d_bussify/4(in4)
  mux2/1 -> d_bussify/3(in3)
  mux1/1 -> d_bussify/2(in2)
  mux0/1 -> d_bussify/1(in1)
  expand1/16(lsb_out1) -> mux15/3
  expand0/16(lsb_out1) -> mux15/2
  sel_expand/16(lsb_out1) -> mux15/1
  expand1/15(out2) -> mux14/3
  expand0/15(out2) -> mux14/2
  sel_expand/15(out2) -> mux14/1
  expand1/14(out3) -> mux13/3
  expand0/14(out3) -> mux13/2
  sel_expand/14(out3) -> mux13/1
  expand1/13(out4) -> mux12/3
  expand0/13(out4) -> mux12/2
  sel_expand/13(out4) -> mux12/1
  expand1/12(out5) -> mux11/3
  expand0/12(out5) -> mux11/2
  sel_expand/12(out5) -> mux11/1
  expand1/11(out6) -> mux10/3
  expand0/11(out6) -> mux10/2
  sel_expand/11(out6) -> mux10/1
  expand1/10(out7) -> mux9/3
  expand0/10(out7) -> mux9/2
  sel_expand/10(out7) -> mux9/1
  expand1/9(out8) -> mux8/3
  expand0/9(out8) -> mux8/2
  sel_expand/9(out8) -> mux8/1
  expand1/8(out9) -> mux7/3
  expand0/8(out9) -> mux7/2
  sel_expand/8(out9) -> mux7/1
  expand1/7(out10) -> mux6/3
  expand0/7(out10) -> mux6/2
  sel_expand/7(out10) -> mux6/1
  expand1/6(out11) -> mux5/3
  expand0/6(out11) -> mux5/2
  sel_expand/6(out11) -> mux5/1
  expand1/5(out12) -> mux4/3
  expand0/5(out12) -> mux4/2
  sel_expand/5(out12) -> mux4/1
  expand1/4(out13) -> mux3/3
  expand0/4(out13) -> mux3/2
  sel_expand/4(out13) -> mux3/1
  expand1/3(out14) -> mux2/3
  expand0/3(out14) -> mux2/2
  sel_expand/3(out14) -> mux2/1
  expand1/2(out15) -> mux1/3
  expand0/2(out15) -> mux1/2
  sel_expand/2(out15) -> mux1/1
  expand1/1(msb_out16) -> mux0/3
  expand0/1(msb_out16) -> mux0/2
  sel_expand/1(msb_out16) -> mux0/1
  d1/1 -> expand1/1(bus_in)
  d0/1 -> expand0/1(bus_in)
  sel/1 -> sel_expand/1(bus_in)

== system rfsoc4x2_ospfb_128/fft_wideband_real1/fft_biplex_real_4x/biplex_core/fft_stage_3/butterfly_direct/shift_replicate ==
  in : Inport
  bussify : Subsystem  AncestorBlock=casper_library_flow_control/bus_create  mask(bus_create){inputNum=16}
      mask prompts: inputNum "Number of inputs:"
      mask init:
      | bus_create_init(gcb,...
      |     'inputNum', inputNum);
  din0_{0..3} (4 alike) : xbsIndex_r4/Delay  rst=off  infoeditControl=Selection of Reset will increase slice count due to use of real FFs and instead of SRLs  en=off  latency=1  reg_retiming=off  dbl_ovrd=off  block_type=delay
  din1_{0..15} (16 alike) : xbsIndex_r4/Delay  rst=off  infoeditControl=Selection of Reset will increase slice count due to use of real FFs and instead of SRLs  en=off  latency=1  reg_retiming=off  dbl_ovrd=off  block_type=delay
  out : Outport
  wires:
  bussify/1(bus_out) -> out/1
  din1_15/1 -> bussify/16(in16)
  din1_14/1 -> bussify/15(in15)
  din1_13/1 -> bussify/14(in14)
  din1_12/1 -> bussify/13(in13)
  din1_11/1 -> bussify/12(in12)
  din1_10/1 -> bussify/11(in11)
  din1_9/1 -> bussify/10(in10)
  din1_8/1 -> bussify/9(in9)
  din1_7/1 -> bussify/8(in8)
  din1_6/1 -> bussify/7(in7)
  din1_5/1 -> bussify/6(in6)
  din1_4/1 -> bussify/5(in5)
  din1_3/1 -> bussify/4(in4)
  din1_2/1 -> bussify/3(in3)
  din1_1/1 -> bussify/2(in2)
  din1_0/1 -> bussify/1(in1)
  din0_3/1 -> din1_15/1, din1_11/1, din1_7/1, din1_3/1
  din0_2/1 -> din1_14/1, din1_10/1, din1_6/1, din1_2/1
  din0_1/1 -> din1_13/1, din1_9/1, din1_5/1, din1_1/1
  din0_0/1 -> din1_12/1, din1_8/1, din1_4/1, din1_0/1
  in/1 -> din0_3/1, din0_2/1, din0_1/1, din0_0/1
